simulink model "GuidanceLaw"  (R2023b)
settings: Solver=ode4  StartTime=0.0  StopTime=400  FixedStep=0.05  RelTol=1e-3
values from neighbouring files (symbols this model uses):
  APCMD_TYPE : value not decoded    [apDataDictionary.sldd]
  missionRoutePlan_struct = struct(      'validWpNum_u8', uint8(5),      'missionRoute_struct', repmat(wpDefault_struct, double(maxWpNum_u8), 1))    [initMissionRoutePlan_MC.m]
  MSSN_TYPE : value not decoded    [apDataDictionary.sldd]
  setPoint_struct = struct('lat_deg_d',double(31.200000),'lon_deg_d',double(121.500000),'alt_m_f',single(100),'yaw_deg_f',single(0))    [APTest.m]
undefined symbols (not defined in the file or in its folder): apParams
libraries: simulink x13, simulink_extras x3
(part 4 of 7)

== matlab function GuidanceLaw/Subsystem/wpMssnHandle/GuiLaw/guiLawSelect/guiLawSelect ==
  data: flightPhase_enum input; guiLawType_u8 output; fwL1LineGui_b output; fwL1CirGui_b output; fwAirSpdGui_b output; fwVertSpdGui_b output; mcSpdGui_b output; yawGui_b output; preWp_struct input; curWp_struct input; segMssnType_u8 output; tiltEnable_b output
function [guiLawType_u8, fwL1LineGui_b, fwL1CirGui_b, fwAirSpdGui_b, fwVertSpdGui_b, mcSpdGui_b, yawGui_b, segMssnType_u8, tiltEnable_b] = guiLawSelect(flightPhase_enum, ...
    preWp_struct, curWp_struct)
%#codegen
%
% 功能：
% 根据当前飞行阶段、上一航点类型和当前航点类型选择导引律。
%
% 当前执行航段定义：
% preWp_struct -> curWp_struct
%
% segMssnType_u8:
% 0：无效，1：旋翼垂直起飞，2：旋翼直线，3：旋翼垂直降落，4：旋翼前倾，5：固定翼后倾，6：固定翼直线，7：固定翼圆弧

%% 获取航点类型

preWpType_u8 = preWp_struct.wpType_u8;
curWpType_u8 = curWp_struct.wpType_u8;

%% 默认关闭所有导引律

guiLawType_u8 = uint8(0);
fwL1LineGui_b = false;
fwL1CirGui_b = false;
fwAirSpdGui_b = false;
fwVertSpdGui_b = false;
mcSpdGui_b = false;
yawGui_b = false;
segMssnType_u8 = uint8(0);    % 航段任务类型无效
tiltEnable_b = false;       % 倾转使能标志

%% 根据上一航点和当前航点判断判断
% 当前是垂直起飞航点
if curWpType_u8 == WP_TYPE.MC_TAKEOFF_WP
    % 旋翼速度导引、偏航角导引使能
    mcSpdGui_b = true;
    yawGui_b = true;
    guiLawType_u8 = uint8(1);
    segMssnType_u8 = uint8(1);        % 航段任务类型为旋翼垂直起飞
    tiltEnable_b = false;

% 当前是旋翼直线航点
elseif (preWpType_u8 == WP_TYPE.MC_TAKEOFF_WP && curWpType_u8 == WP_TYPE.MC_LINE_WP) || ...
        (preWpType_u8 == WP_TYPE.FW_LINE_WP && curWpType_u8 == WP_TYPE.MC_LINE_WP)||...
        (preWpType_u8 == WP_TYPE.MC_LINE_WP && curWpType_u8 == WP_TYPE.MC_LINE_WP)
    switch flightPhase_enum
        case FLIGHT_PHASE.MC_FLIGHT
            % 旋翼速度导引、偏航角导引使能
            mcSpdGui_b = true;
            yawGui_b = true;
            guiLawType_u8 = uint8(1);
            segMssnType_u8 = uint8(2);        % 航段任务类型为旋翼直线

        case FLIGHT_PHASE.TILT_FLIGHT
            % L1直线导引、fw空速导引、fw垂速导引、偏航角导引使能
            fwL1LineGui_b = true;
            fwAirSpdGui_b = true;
            fwVertSpdGui_b = true;
            yawGui_b = true;
            guiLawType_u8 = uint8(2);
            segMssnType_u8 = uint8(5);        % 航段任务类型为固定翼后倾

        case FLIGHT_PHASE.FW_FLIGHT
            % L1直线导引、fw空速导引、fw垂速导引使能
            fwL1LineGui_b = true;
            fwAirSpdGui_b = true;
            fwVertSpdGui_b = true;
            guiLawType_u8 = uint8(3);
            segMssnType_u8 = uint8(5);        % 航段任务类型为固定翼后倾

        otherwise
            % 不处理
    end
    tiltEnable_b = false;

% 当前是垂直降落航点
elseif (preWpType_u8 == WP_TYPE.MC_TAKEOFF_WP && curWpType_u8 == WP_TYPE.MC_LAND_WP) || (preWpType_u8 == WP_TYPE.FW_LINE_WP && curWpType_u8 == WP_TYPE.MC_LAND_WP)||...
        (preWpType_u8 == WP_TYPE.MC_LINE_WP && curWpType_u8 == WP_TYPE.MC_LAND_WP) || (preWpType_u8 == WP_TYPE.MC_LAND_WP && curWpType_u8 == WP_TYPE.MC_LAND_WP)
    switch flightPhase_enum
        case {FLIGHT_PHASE.MC_FLIGHT, FLIGHT_PHASE.MC_GROUND}
            % 旋翼速度导引、偏航角导引使能
            mcSpdGui_b = true;
            yawGui_b = true;
            guiLawType_u8 = uint8(1);

            if preWpType_u8 == WP_TYPE.MC_LAND_WP && curWpType_u8 == WP_TYPE.MC_LAND_WP
                segMssnType_u8 = uint8(3);        % 航段任务类型为旋翼垂直着陆
            else
                segMssnType_u8 = uint8(2);        % 航段任务类型为旋翼直线
            end

        case FLIGHT_PHASE.TILT_FLIGHT
            % L1直线导引、fw空速导引、fw垂速导引、偏航角导引使能
            fwL1LineGui_b = true;
            fwAirSpdGui_b = true;
            fwVertSpdGui_b = true;
            yawGui_b = true;
            guiLawType_u8 = uint8(2);
            segMssnType_u8 = uint8(5);        % 航段任务类型为固定翼后倾

        case FLIGHT_PHASE.FW_FLIGHT
            % L1直线导引、fw空速导引、fw垂速导引使能
            fwL1LineGui_b = true;
            fwAirSpdGui_b = true;
            fwVertSpdGui_b = true;
            guiLawType_u8 = uint8(3);
            segMssnType_u8 = uint8(5);        % 航段任务类型为固定翼后倾

        otherwise
            % 不处理
    end
    tiltEnable_b = false;
    
% 当前是固定翼直线航点
elseif (preWpType_u8 == WP_TYPE.MC_TAKEOFF_WP && curWpType_u8 == WP_TYPE.FW_LINE_WP) || (preWpType_u8 == WP_TYPE.MC_LINE_WP && curWpType_u8 == WP_TYPE.FW_LINE_WP)||...
        (preWpType_u8 == WP_TYPE.FW_LINE_WP && curWpType_u8 == WP_TYPE.FW_LINE_WP)
    switch flightPhase_enum
        case {FLIGHT_PHASE.MC_FLIGHT, FLIGHT_PHASE.TILT_FLIGHT}
            % L1直线导引、fw空速导引、fw垂速导引、偏航角导引使能
            fwL1LineGui_b = true;
            fwAirSpdGui_b = true;
            fwVertSpdGui_b = true;
            yawGui_b = true;
            guiLawType_u8 = uint8(2);
            segMssnType_u8 = uint8(4);        % 航段任务类型为旋翼前倾

        case FLIGHT_PHASE.FW_FLIGHT
            % L1直线导引、fw空速导引、fw垂速导引使能
            fwL1LineGui_b = true;
            fwAirSpdGui_b = true;
            fwVertSpdGui_b = true;
            guiLawType_u8 = uint8(3);
            segMssnType_u8 = uint8(6);        % 航段任务类型为固定翼直线

        otherwise
            % 不处理
    end
    tiltEnable_b = true;

% 当前是圆弧航点
elseif curWpType_u8 == WP_TYPE.FW_CIR_WP
    % L1圆弧导引、fw空速导引、fw垂速导引使能
    fwL1CirGui_b = true;
    fwAirSpdGui_b = true;
    fwVertSpdGui_b = true;
    guiLawType_u8 = uint8(4);
    tiltEnable_b = true;
    segMssnType_u8 = uint8(7);        % 航段任务类型为固定翼圆弧

else
    % 不处理
end

end

== matlab function GuidanceLaw/Subsystem/wpMssnHandle/GuiLaw/fwAirSpdGuidance/fwAirSpdGuidance ==
  data: curPosNEU_m_f input; curAirSpd_mps_f input; velNEU_mps_f input; preWp_struct input; speedCmd_mps_f output; curWp_struct input; dt_s_f input; reset_b input; param_f input; segMssnType_u8 input; mssnType_u8 input
function speedCmd_mps_f = fwAirSpdGuidance(curPosNEU_m_f, curAirSpd_mps_f, velNEU_mps_f, preWp_struct, curWp_struct, dt_s_f, reset_b, param_f, segMssnType_u8, mssnType_u8)
%#codegen
%
% 速度指令生成导引算法
%
% 功能：
% 1. 前倾和固定翼飞行阶段生成等效空速指令；
% 2. 后倾阶段生成水平地速指令；
% 3. 普通自动后倾根据目标点剩余沿程距离生成减速包线；
% 4. 自动着陆定向后倾进入航段后立即按设定减速度降低水平速度；
% 5. 定向后倾目标点只用于航向/航迹锚定，不参与速度指令计算；
% 6. 后倾速度降至旋翼阶段准入速度后，由外部切换至旋翼导引律。
%
% param_f定义：
% 1  minOptAirspeed_mps_f          正常固定翼最小空速，m/s；
% 2  maxOptAirSpeed_mps_f          最大速度，m/s；
% 3  cruiseAirspeed_mps_f          默认巡航空速，m/s；
% 4  airspeedAccelMax_mps2_f       空速指令最大增加率，m/s^2；
% 5  airspeedDecelMax_mps2_f       空速指令最大减小率，m/s^2；
% 6  backTransDecel_mps2_f         后倾期望水平减速度，m/s^2；
% 7  backTransAnchorRadius_m_f     普通自动后倾减速包线锚定半径，m；
% 8  backTransFastAnchorSpd_mps_f  普通自动后倾快速过点虚拟末速度，m/s；
%                                  同时作为定向后倾目标水平速度，m/s。
%
% 注意：
% 当该函数用于自动着陆定向后倾时，param_f(8)应低于外部MC_FLIGHT
% 准入速度，并留有适当裕度。
% 当前简化六自由度模型在水平速度不大于10 m/s时进入MC_FLIGHT，
% 因此建议本参数使用7~8 m/s。

persistent initialized_b
persistent backTransLast_b
% persistent directionBackTiltLast_b
persistent speedCmdState_mps_f

if isempty(initialized_b)
    initialized_b = false;
    backTransLast_b = false;
    % directionBackTiltLast_b = false;
    speedCmdState_mps_f = single(0.0);
end

%% 1. 参数解析

minOptAirspeed_mps_f = max(param_f(1), single(0.0));
maxOptAirspeed_mps_f = max(param_f(2), minOptAirspeed_mps_f);

cruiseAirspeed_mps_f = max(param_f(3), single(0.0));

airspeedAccelMax_mps2_f = max(param_f(4), single(0.0));
airspeedDecelMax_mps2_f = max(param_f(5), single(0.0));

backTransDecel_mps2_f = max(param_f(6), single(0.1));
backTransAnchorRadius_m_f = max(param_f(7), single(0.0));
backTransFastAnchorSpd_mps_f = max(param_f(8), single(0.0));

% 定向后倾复用param_f(8)作为目标水平速度。该速度允许低于正常固定翼
% 最小空速，因为后倾过程中旋翼升力逐步接管。
% directionBackTiltTargetSpd_mps_f = constrain_scalar(max(param_f(8), single(0.0)), single(0.0), maxOptAirspeed_mps_f);

dtUse_s_f = max(dt_s_f, single(0.0));

%% 2. 判断速度导引模式

isBackTransition_b = segMssnType_u8 == uint8(5);        % 后倾航段任务
isDirectionBackTilt_b = isBackTransition_b && mssnType_u8 == MSSN_TYPE.AUTO_LAND_DIRECTION_BACK_TILT;

speedModeChanged_b = isBackTransition_b ~= backTransLast_b; %|| isDirectionBackTilt_b ~= directionBackTiltLast_b;

%% 3. 正常固定翼空速导引

if ~isBackTransition_b

    airSpdPlan_mps_f = curWp_struct.spd_mps_f;

    if airSpdPlan_mps_f > single(0.0)
        speedBase_mps_f = airSpdPlan_mps_f;
    else
        speedBase_mps_f = cruiseAirspeed_mps_f;
    end

    speedRaw_mps_f = constrain_scalar(speedBase_mps_f, minOptAirspeed_mps_f, maxOptAirspeed_mps_f);

    if reset_b || ~initialized_b || speedModeChanged_b

        % 从当前实际空速无跳变接入正常固定翼空速导引。
        speedCmdState_mps_f = constrain_scalar(curAirSpd_mps_f, minOptAirspeed_mps_f, maxOptAirspeed_mps_f);

        initialized_b = true;

    else

        speedCmdState_mps_f = rateLimit(speedRaw_mps_f, speedCmdState_mps_f, airspeedAccelMax_mps2_f, airspeedDecelMax_mps2_f, dtUse_s_f);

        speedCmdState_mps_f = constrain_scalar(speedCmdState_mps_f, minOptAirspeed_mps_f, maxOptAirspeed_mps_f);

    end

%% 4. 后倾阶段水平地速导引

else

    %% 4.1 计算当前水平地速

    groundSpdSq_m2ps2_f = velNEU_mps_f(1) * velNEU_mps_f(1) + velNEU_mps_f(2) * velNEU_mps_f(2);

    groundSpd_mps_f = sqrt(max(groundSpdSq_m2ps2_f, single(0.0)));

    if isDirectionBackTilt_b

        %% 4.2 自动着陆定向后倾：进入航段后立即减速

        if reset_b || ~initialized_b || speedModeChanged_b

            % 从当前实际水平地速无跳变接入。
            speedCmdState_mps_f = constrain_scalar(groundSpd_mps_f, single(0.0), maxOptAirspeed_mps_f);

            initialized_b = true;

        else

            % 不计算锚点距离。锚点只供横向航迹导引使用。
            speedCmdState_mps_f = rateLimit(single(0), speedCmdState_mps_f, single(0.0), backTransDecel_mps2_f, dtUse_s_f);

            % 定向后倾阶段不施加正常固定翼最小空速下限。
            speedCmdState_mps_f = constrain_scalar(speedCmdState_mps_f, single(0), maxOptAirspeed_mps_f);

        end

    else

        %% 4.3 普通自动后倾：保留原来的距离减速包线

        %% 4.3.1 计算水平航段向量

        pathVectorN_m_f = curWp_struct.posN_m_f - preWp_struct.posN_m_f;
        pathVectorE_m_f = curWp_struct.posE_m_f - preWp_struct.posE_m_f;

        pathLengthSq_m2_f = pathVectorN_m_f * pathVectorN_m_f + pathVectorE_m_f * pathVectorE_m_f;

        pathLength_m_f = sqrt(max(pathLengthSq_m2_f, single(0.0)));

        %% 4.3.2 计算当前位置到目标航点的向量

        targetVectorN_m_f = curWp_struct.posN_m_f - curPosNEU_m_f(1);
        targetVectorE_m_f = curWp_struct.posE_m_f - curPosNEU_m_f(2);

        targetDistSq_m2_f = targetVectorN_m_f * targetVectorN_m_f + targetVectorE_m_f * targetVectorE_m_f;

        targetDist_m_f = sqrt(max(targetDistSq_m2_f, single(0.0)));

        %% 4.3.3 计算剩余沿程距离

        if pathLength_m_f > single(0.1)

            pathTangentN_f = pathVectorN_m_f / pathLength_m_f;
            pathTangentE_f = pathVectorE_m_f / pathLength_m_f;

            remainAlongTrack_m_f = targetVectorN_m_f * pathTangentN_f + targetVectorE_m_f * pathTangentE_f;

        else

            remainAlongTrack_m_f = targetDist_m_f;

        end

        remainAlongTrack_m_f = max(remainAlongTrack_m_f, single(0.0));

        %% 4.3.4 确定普通自动后倾虚拟末速度

        if curWp_struct.fastWp_b
            speedAnchor_mps_f = backTransFastAnchorSpd_mps_f;       % 这里给了个旋翼最大巡航速度
        else
            speedAnchor_mps_f = single(0.0);
        end

        %% 4.3.5 根据剩余距离反算速度包线

        effectiveRemainDist_m_f = remainAlongTrack_m_f - backTransAnchorRadius_m_f;

        effectiveRemainDist_m_f = max(effectiveRemainDist_m_f, single(0.0));

        envelopeSpdSq_m2ps2_f = speedAnchor_mps_f * speedAnchor_mps_f + single(2.0) * backTransDecel_mps2_f * effectiveRemainDist_m_f;

        groundSpdEnvelopeRaw_mps_f = sqrt(max(envelopeSpdSq_m2ps2_f, single(0.0)));

        groundSpdEnvelope_mps_f = constrain_scalar(groundSpdEnvelopeRaw_mps_f, minOptAirspeed_mps_f, maxOptAirspeed_mps_f);

        %% 4.3.6 更新普通自动后倾速度指令

        if reset_b || ~initialized_b || speedModeChanged_b

            speedCmdState_mps_f = constrain_scalar(groundSpd_mps_f, minOptAirspeed_mps_f, maxOptAirspeed_mps_f);

            initialized_b = true;

        else

            speedRaw_mps_f = min(speedCmdState_mps_f, groundSpdEnvelope_mps_f);

            speedCmdState_mps_f = rateLimit(speedRaw_mps_f, speedCmdState_mps_f, single(0.0), backTransDecel_mps2_f, dtUse_s_f);

            speedCmdState_mps_f = constrain_scalar(speedCmdState_mps_f, minOptAirspeed_mps_f, maxOptAirspeed_mps_f);

        end

    end

end


%% 5. 输出及模式记录

speedCmd_mps_f = speedCmdState_mps_f;

backTransLast_b = isBackTransition_b;
% directionBackTiltLast_b = isDirectionBackTilt_b;

end

== matlab function GuidanceLaw/Subsystem/wpMssnHandle/GuiLaw/fwAirSpdGuidance/fwAirSpdGuidance1 ==
  data: curPosNEU_m_f input; curAirSpd_mps_f input; velNEU_mps_f input; preWp_struct input; speedCmd_mps_f output; curWp_struct input; dt_s_f input; reset_b input; param_f input; segMssnType_u8 input
function speedCmd_mps_f = fwAirSpdGuidance(curPosNEU_m_f, curAirSpd_mps_f, velNEU_mps_f, preWp_struct, curWp_struct, dt_s_f, reset_b, param_f, segMssnType_u8)
%#codegen
%
% 速度指令生成导引算法
%
% 功能：
% 1. 前倾和固定翼飞行阶段生成等效空速指令；
% 2. 后倾阶段生成水平地速指令；
% 3. 后倾阶段根据剩余沿程距离反算允许水平地速；
% 4. 快速过点采用非零虚拟末速度构造减速包线；
% 5. 减速悬停采用零虚拟末速度构造减速包线；
% 6. 完成旋翼构型转换后，由外部切换至旋翼导引律。
%
% param_f定义：
% 1  minOptAirspeed_mps_f          最小空速，m/s；
% 2  maxOptAirSpeed_mps_f          最大速度，m/s；
% 3  cruiseAirspeed_mps_f          默认巡航空速，m/s；
% 4  airspeedAccelMax_mps2_f       空速指令最大增加率，m/s^2；
% 5  airspeedDecelMax_mps2_f       空速指令最大减小率，m/s^2；
% 6  backTransDecel_mps2_f         后倾期望水平减速度，m/s^2；
% 7  backTransAnchorRadius_m_f     后倾减速包线锚定半径，m；
% 8  backTransFastAnchorSpd_mps_f  快速过点虚拟末速度锚点，m/s。

persistent initialized_b
persistent backTransLast_b
persistent speedCmdState_mps_f

if isempty(initialized_b)
    initialized_b = false;
    backTransLast_b = false;
    speedCmdState_mps_f = single(0.0);
end

%% 1. 参数解析

minOptAirspeed_mps_f = max(param_f(1), single(0.0));
maxOptAirspeed_mps_f = max(param_f(2), minOptAirspeed_mps_f);

cruiseAirspeed_mps_f = max(param_f(3), single(0.0));

airspeedAccelMax_mps2_f = max(param_f(4), single(0.0));
airspeedDecelMax_mps2_f = max(param_f(5), single(0.0));

backTransDecel_mps2_f = max(param_f(6), single(0.1));
backTransAnchorRadius_m_f = max(param_f(7), single(0.0));
backTransFastAnchorSpd_mps_f = max(param_f(8), single(0.0));

dtUse_s_f = max(dt_s_f, single(0.0));

%% 2. 判断速度导引模式

isBackTransition_b = segMssnType_u8 == uint8(5);
speedModeChanged_b = isBackTransition_b ~= backTransLast_b;

%% 3. 正常固定翼空速导引

if ~isBackTransition_b

    airSpdPlan_mps_f = curWp_struct.spd_mps_f;

    if airSpdPlan_mps_f > single(0.0)
        speedBase_mps_f = airSpdPlan_mps_f;
    else
        speedBase_mps_f = cruiseAirspeed_mps_f;
    end

    speedRaw_mps_f = constrain_scalar(speedBase_mps_f, minOptAirspeed_mps_f, maxOptAirspeed_mps_f);

    if reset_b || ~initialized_b || speedModeChanged_b

        % 从当前实际空速接入固定翼空速导引。
        speedCmdState_mps_f = constrain_scalar(curAirSpd_mps_f, minOptAirspeed_mps_f, maxOptAirspeed_mps_f);
        initialized_b = true;

    else

        speedCmdState_mps_f = rateLimit(speedRaw_mps_f, speedCmdState_mps_f, airspeedAccelMax_mps2_f, airspeedDecelMax_mps2_f, dtUse_s_f);

        speedCmdState_mps_f = constrain_scalar(speedCmdState_mps_f, minOptAirspeed_mps_f, maxOptAirspeed_mps_f);

    end

%% 4. 后倾阶段水平地速导引

else

    %% 4.1 计算当前水平地速

    groundSpdSq_m2ps2_f = velNEU_mps_f(1) * velNEU_mps_f(1) + velNEU_mps_f(2) * velNEU_mps_f(2);

    groundSpd_mps_f = sqrt(max(groundSpdSq_m2ps2_f, single(0.0)));

    %% 4.2 计算水平航段向量

    pathVectorN_m_f = curWp_struct.posN_m_f - preWp_struct.posN_m_f;
    pathVectorE_m_f = curWp_struct.posE_m_f - preWp_struct.posE_m_f;

    pathLengthSq_m2_f = pathVectorN_m_f * pathVectorN_m_f + pathVectorE_m_f * pathVectorE_m_f;

    pathLength_m_f = sqrt(max(pathLengthSq_m2_f, single(0.0)));

    %% 4.3 计算当前位置到目标航点的向量

    targetVectorN_m_f = curWp_struct.posN_m_f - curPosNEU_m_f(1);
    targetVectorE_m_f = curWp_struct.posE_m_f - curPosNEU_m_f(2);

    targetDistSq_m2_f = targetVectorN_m_f * targetVectorN_m_f + targetVectorE_m_f * targetVectorE_m_f;

    targetDist_m_f = sqrt(max(targetDistSq_m2_f, single(0.0)));

    %% 4.4 计算剩余沿程距离

    if pathLength_m_f > single(0.5)

        pathTangentN_f = pathVectorN_m_f / pathLength_m_f;
        pathTangentE_f = pathVectorE_m_f / pathLength_m_f;

        remainAlongTrack_m_f = targetVectorN_m_f * pathTangentN_f + targetVectorE_m_f * pathTangentE_f;

    else

        % 航段长度过小时退化为目标点直线距离。
        remainAlongTrack_m_f = targetDist_m_f;

    end

    remainAlongTrack_m_f = max(remainAlongTrack_m_f, single(0.0));

    %% 4.5 确定虚拟末速度锚点

    if curWp_struct.fastWp_b
    
        % 非零虚拟末速度锚点。
        speedAnchor_mps_f = backTransFastAnchorSpd_mps_f;
    
    else
    
        % 零虚拟末速度锚点。
        speedAnchor_mps_f = single(0.0);
    
    end

    %% 4.6 根据剩余距离反算速度包线

    effectiveRemainDist_m_f = remainAlongTrack_m_f - backTransAnchorRadius_m_f;

    effectiveRemainDist_m_f = max(effectiveRemainDist_m_f, single(0.0));

    envelopeSpdSq_m2ps2_f = speedAnchor_mps_f * speedAnchor_mps_f + single(2.0) * backTransDecel_mps2_f * effectiveRemainDist_m_f;

    groundSpdEnvelopeRaw_mps_f = sqrt(max(envelopeSpdSq_m2ps2_f, single(0.0)));

    groundSpdEnvelope_mps_f = constrain_scalar(groundSpdEnvelopeRaw_mps_f, minOptAirspeed_mps_f, maxOptAirspeed_mps_f);

    %% 4.7 更新后倾速度指令状态

    if reset_b || ~initialized_b || speedModeChanged_b
    
        speedCmdState_mps_f = constrain_scalar(groundSpd_mps_f, minOptAirspeed_mps_f, maxOptAirspeed_mps_f);
    
        initialized_b = true;
    
    else
    
        speedRaw_mps_f = min(speedCmdState_mps_f, groundSpdEnvelope_mps_f);
    
        speedCmdState_mps_f = rateLimit(speedRaw_mps_f, speedCmdState_mps_f, single(0.0), backTransDecel_mps2_f, dtUse_s_f);
    
        speedCmdState_mps_f = constrain_scalar(speedCmdState_mps_f, minOptAirspeed_mps_f, maxOptAirspeed_mps_f);
    
    end

end

%% 5. 输出及模式记录

speedCmd_mps_f = speedCmdState_mps_f;

backTransLast_b = isBackTransition_b;

end

== matlab function GuidanceLaw/Subsystem/wpMssnHandle/GuiLaw/mcSpdGuidance/mcTrajectoryGeneratorNEU/TrajectoryGeneratorNEU1 ==
  data: trajPosNEU_m_f output; curPosNEU_m_f input; curVelNEU_mps_f input; curAccNEU_mps2_f input; preWpNEU_m_f input; curWpNEU_m_f input; nextWpNEU_m_f input; velSpNEU_mps_f input; posVelValid_vec input; isHoverWp_b input; forceStop_b input; segSwitch_b input; newOriOldNEU_m_f input; dt_s_f input; reset_b input; paramNE_f input; trajVelNEU_mps_f output; trajAccNEU_mps2_f output; trajJerkNEU_mps3_f output; paramU_f input
function [trajPosNEU_m_f, trajVelNEU_mps_f, trajAccNEU_mps2_f, trajJerkNEU_mps3_f] = trajGeneratorNEU(curPosNEU_m_f, curVelNEU_mps_f, curAccNEU_mps2_f, preWpNEU_m_f, curWpNEU_m_f, nextWpNEU_m_f, ...
    velSpNEU_mps_f, posVelValid_vec, isHoverWp_b, forceStop_b, segSwitch_b, newOriOldNEU_m_f, dt_s_f, reset_b, paramNE_f, paramU_f)
%#codegen
%
% 功能：
% 生成NEU三轴jerk受限平滑轨迹，并进行N/E/U三轴S曲线时间同步。
%
% velSpNEU_mps_f：
% 1. 对应位置无效时，为纯速度目标；
% 2. 对应位置有效时，为位置导引速度上的速度前馈。
%
% posVelValid_vec：[posNEValid; velNEValid; posUValid; velUValid]
%
% paramNE_f：
% 1 最大水平jerk，[m/s^3]
% 2 最大水平加速度，[m/s^2]
% 3 最大水平速度，[m/s]
% 4 水平巡航速度，[m/s]
% 5 最大允许水平轨迹误差，[m]
% 6 水平航点接受半径，[m]
% 7 最小前视距离，[m]
% 8 转弯判断最小轨迹速度，[m/s]
% 9 转弯判断方向余弦阈值
% 10 前倾转换阶段旋翼水平速度，[m/s]
%
% paramU_f：
% 1 最大垂向jerk，[m/s^3]
% 2 爬升轨迹使用的最大垂向加速度幅值，[m/s^2]
% 3 下降轨迹使用的最大垂向加速度幅值，[m/s^2]
% 4 最大爬升速度，[m/s]
% 5 最大下降速度幅值，[m/s]
% 6 最大允许垂向轨迹误差，[m]
% 7 垂向航点接受半径，[m]
%
% 垂向非对称约束：
% 1. 根据未平滑垂向速度目标rawVelSpNEU_mps_f(3)的方向，选择一整套
%    垂向速度和加速度幅值约束；
% 2. 选定后，单轴S曲线规划器内部仍使用对称的+/-maxAcceleration约束；
% 3. rawVelSpU为0时保持上一套约束，避免停车附近反复切换。

%% 常量

smallValue_f = single(1.0e-6);
floatEpsilon_f = single(1.1920929e-7);
clampAccuracy_mps_f = single(0.5);

%% 最小持久状态
% 轨迹生成器每个周期都会根据当前状态重新规划S曲线，并在同一周期推进dt。
persistent trajAccStateNEU_mps2_f trajVelStateNEU_mps_f trajPosStateNEU_m_f
persistent selectedUConstraintModeState_i8
persistent previousMaxSpeedNEState_mps_f
persistent initialized_b

if isempty(initialized_b)
    initialized_b = false;

    trajAccStateNEU_mps2_f = single(zeros(3,1));
    trajVelStateNEU_mps_f = single(zeros(3,1));
    trajPosStateNEU_m_f = single(zeros(3,1));
    selectedUConstraintModeState_i8 = int8(0);
    previousMaxSpeedNEState_mps_f = single(0.0);
else
    initialized_b = true;
end

%% 参数读取
maxJerkNE_mps3_f = max(paramNE_f(1), smallValue_f);
maxAccNE_mps2_f = max(paramNE_f(2), smallValue_f);
maxVelNE_mps_f = max(paramNE_f(3), smallValue_f);
cruiseSpeedNE_mps_f = constrain_scalar(paramNE_f(4), single(0.0), maxVelNE_mps_f);
maxTrajErrorNE_m_f = max(paramNE_f(5), smallValue_f);
horizonAptRadius_m_f = max(paramNE_f(6), smallValue_f);
minLookaheadDist_m_f = max(paramNE_f(7), horizonAptRadius_m_f);
turnMinSpeed_mps_f = max(paramNE_f(8), single(0.0));
turnCosThreshold_f = constrain_scalar(paramNE_f(9), single(-1.0), single(1.0));
fwdFixedSpd_mps_f = max(paramNE_f(10), smallValue_f);

maxJerkU_mps3_f = max(paramU_f(1), smallValue_f);
maxAccUp_mps2_f = max(paramU_f(2), smallValue_f);
maxAccDown_mps2_f = max(paramU_f(3), smallValue_f);
maxVelUp_mps_f = max(paramU_f(4), smallValue_f);
maxVelDown_mps_f = max(paramU_f(5), smallValue_f);
maxTrajErrorU_m_f = max(paramU_f(6), smallValue_f);
verticalAcceptanceRadius_m_f = max(paramU_f(7), smallValue_f);

axisMaxJerkNEU_mps3_f = single([maxJerkNE_mps3_f; maxJerkNE_mps3_f; maxJerkU_mps3_f]);

dtEff_s_f = max(dt_s_f, single(0.0));

%% 输入有效性
posNEValid_b = logical(posVelValid_vec(1));
velNEValid_b = logical(posVelValid_vec(2));
posUValid_b = logical(posVelValid_vec(3));
velUValid_b = logical(posVelValid_vec(4));

%% 初始化、复位或航段坐标系切换
if reset_b || ~initialized_b
    trajAccStateNEU_mps2_f = curAccNEU_mps2_f;
    trajVelStateNEU_mps_f = curVelNEU_mps_f;
    trajPosStateNEU_m_f = curPosNEU_m_f;

    trajAccStateNEU_mps2_f(1) = constrain_scalar(curAccNEU_mps2_f(1), -maxAccNE_mps2_f, maxAccNE_mps2_f);
    trajAccStateNEU_mps2_f(2) = constrain_scalar(curAccNEU_mps2_f(2), -maxAccNE_mps2_f, maxAccNE_mps2_f);
    trajAccStateNEU_mps2_f(3) = constrain_scalar(curAccNEU_mps2_f(3), -maxAccDown_mps2_f, maxAccUp_mps2_f);

    trajVelStateNEU_mps_f(1) = constrain_scalar(curVelNEU_mps_f(1), -maxVelNE_mps_f, maxVelNE_mps_f);
    trajVelStateNEU_mps_f(2) = constrain_scalar(curVelNEU_mps_f(2), -maxVelNE_mps_f, maxVelNE_mps_f);
    trajVelStateNEU_mps_f(3) = constrain_scalar(curVelNEU_mps_f(3), -maxVelDown_mps_f, maxVelUp_mps_f);

    % 1表示爬升约束，-1表示下降约束，0表示尚未选择方向并采用保守值。
    if curVelNEU_mps_f(3) > smallValue_f
        selectedUConstraintModeState_i8 = int8(1);
    elseif curVelNEU_mps_f(3) < -smallValue_f
        selectedUConstraintModeState_i8 = int8(-1);
    else
        selectedUConstraintModeState_i8 = int8(0);
    end

    previousMaxSpeedNEState_mps_f = single(0.0);

elseif segSwitch_b
    % 各航段坐标轴方向不变，仅平移原点
    trajPosStateNEU_m_f = trajPosStateNEU_m_f - newOriOldNEU_m_f;
else
    % 不处理
end

%% 按有效性组合生成原始速度目标

% 先装载速度输入。位置有效时，它是位置速度的前馈；位置无效时，
% 它就是直接送给S曲线平滑器的纯速度目标。无效速度分量保持为0。
rawVelSpNEU_mps_f = single(zeros(3,1));

if velNEValid_b
    rawVelSpNEU_mps_f(1:2) = velSpNEU_mps_f(1:2);
end

if velUValid_b
    rawVelSpNEU_mps_f(3) = velSpNEU_mps_f(3);
end

if forceStop_b
    % 强制停车优先级最高，忽略位置目标和速度前馈。
    rawVelSpNEU_mps_f = single(zeros(3,1));

elseif posNEValid_b && posUValid_b
    %% NE和U位置同时有效：生成三维位置速度目标
    waypointsNEU_m_f = [preWpNEU_m_f, curWpNEU_m_f, nextWpNEU_m_f];

    [crossingPointNEU_m_f, targetSpeedNE_mps_f, previousMaxSpeedNEState_mps_f] = get_xy_guidance_constraints_handle(trajPosStateNEU_m_f, trajVelStateNEU_mps_f, waypointsNEU_m_f, ...
        isHoverWp_b, cruiseSpeedNE_mps_f, maxJerkNE_mps3_f, maxAccNE_mps2_f, horizonAptRadius_m_f, minLookaheadDist_m_f, turnMinSpeed_mps_f, ...
        turnCosThreshold_f, previousMaxSpeedNEState_mps_f, smallValue_f);

    if isHoverWp_b
        nextWpForUSpeed_m_f = curWpNEU_m_f(3);
    else
        nextWpForUSpeed_m_f = nextWpNEU_m_f(3);
    end

    maxAllowedSpeedU_mps_f = get_max_z_speed_handle(trajPosStateNEU_m_f(3), curWpNEU_m_f(3), nextWpForUSpeed_m_f, maxJerkU_mps3_f, maxAccUp_mps2_f, maxAccDown_mps2_f, ...
        maxVelUp_mps_f, maxVelDown_mps_f, verticalAcceptanceRadius_m_f, smallValue_f);

    posToCrossingNEU_m_f = crossingPointNEU_m_f - trajPosStateNEU_m_f;
    directionToCrossingNEU_f = unit_or_zero(posToCrossingNEU_m_f, smallValue_f);
    combinedSpeed_mps_f = sqrt(targetSpeedNE_mps_f * targetSpeedNE_mps_f + maxAllowedSpeedU_mps_f * maxAllowedSpeedU_mps_f);
    posVelSpNEU_mps_f = directionToCrossingNEU_f * combinedSpeed_mps_f;

    % 先限制水平模长，再限制垂向模长。
    % 0.5是小速度区间判定精度accuracy，不是另一方向的固定缩放系数。
    posVelSpNEU_mps_f = clamp_to_xy_norm(posVelSpNEU_mps_f, targetSpeedNE_mps_f, clampAccuracy_mps_f, floatEpsilon_f);
    posVelSpNEU_mps_f = clamp_to_u_norm(posVelSpNEU_mps_f, maxAllowedSpeedU_mps_f, clampAccuracy_mps_f, floatEpsilon_f);

    if velNEValid_b
        rawVelSpNEU_mps_f(1:2) = rawVelSpNEU_mps_f(1:2) + posVelSpNEU_mps_f(1:2);
    else
        rawVelSpNEU_mps_f(1:2) = posVelSpNEU_mps_f(1:2);
    end

    if velUValid_b
        rawVelSpNEU_mps_f(3) = rawVelSpNEU_mps_f(3) + posVelSpNEU_mps_f(3);
    else
        rawVelSpNEU_mps_f(3) = posVelSpNEU_mps_f(3);
    end

elseif posNEValid_b
    %% 仅NE位置有效：生成二维水平位置速度目标
    waypointsNEU_m_f = [preWpNEU_m_f, curWpNEU_m_f, nextWpNEU_m_f];

    [crossingPointNEU_m_f, targetSpeedNE_mps_f, previousMaxSpeedNEState_mps_f] = get_xy_guidance_constraints_handle(trajPosStateNEU_m_f, trajVelStateNEU_mps_f, waypointsNEU_m_f, ...
        isHoverWp_b, cruiseSpeedNE_mps_f, maxJerkNE_mps3_f, maxAccNE_mps2_f, horizonAptRadius_m_f, minLookaheadDist_m_f, turnMinSpeed_mps_f, ...
        turnCosThreshold_f, previousMaxSpeedNEState_mps_f, smallValue_f);

    posToCrossingNE_m_f = crossingPointNEU_m_f(1:2) - trajPosStateNEU_m_f(1:2);
    directionToCrossingNE_f = unit_or_zero(posToCrossingNE_m_f, smallValue_f);
    posVelSpNE_mps_f = directionToCrossingNE_f * targetSpeedNE_mps_f;

    if velNEValid_b
        rawVelSpNEU_mps_f(1:2) = rawVelSpNEU_mps_f(1:2) + posVelSpNE_mps_f;
    else
        rawVelSpNEU_mps_f(1:2) = posVelSpNE_mps_f;
    end

elseif posUValid_b
    %% 仅U位置有效：生成一维垂向位置速度目标
    if isHoverWp_b
        nextWpForUSpeed_m_f = curWpNEU_m_f(3);
    else
        nextWpForUSpeed_m_f = nextWpNEU_m_f(3);
    end

    maxAllowedSpeedU_mps_f = get_max_z_speed_handle(trajPosStateNEU_m_f(3), curWpNEU_m_f(3), nextWpForUSpeed_m_f, maxJerkU_mps3_f, maxAccUp_mps2_f, maxAccDown_mps2_f, ...
        maxVelUp_mps_f, maxVelDown_mps_f, verticalAcceptanceRadius_m_f, smallValue_f);

    posErrorU_m_f = curWpNEU_m_f(3) - trajPosStateNEU_m_f(3);
    posVelSpU_mps_f = single(0.0);

    if abs(posErrorU_m_f) > smallValue_f
        posVelSpU_mps_f = sign(posErrorU_m_f) * maxAllowedSpeedU_mps_f;
    end

    if velUValid_b
        rawVelSpNEU_mps_f(3) = rawVelSpNEU_mps_f(3) + posVelSpU_mps_f;
    else
        rawVelSpNEU_mps_f(3) = posVelSpU_mps_f;
    end

else
    % 不处理，直接使用前馈速度
end

% 位置速度和速度前馈相加后，统一执行最终性能包线保护。
rawVelSpNEU_mps_f(1:2) = limit_vector_2d(rawVelSpNEU_mps_f(1:2), maxVelNE_mps_f, smallValue_f);     % 超长放缩
rawVelSpNEU_mps_f(3) = constrain_scalar(rawVelSpNEU_mps_f(3), -maxVelDown_mps_f, maxVelUp_mps_f);

%% 选择当前垂向整套约束
% NEU中U向上为正：rawVelSpU>0选择爬升约束，rawVelSpU<0选择下降约束。
if rawVelSpNEU_mps_f(3) > smallValue_f
    selectedUConstraintModeState_i8 = int8(1);
elseif rawVelSpNEU_mps_f(3) < -smallValue_f
    selectedUConstraintModeState_i8 = int8(-1);
else
    % 保持上一周期所选模式，使停车S曲线沿用进入停车前的整套参数。
end

if selectedUConstraintModeState_i8 > int8(0)
    selectedMaxAccU_mps2_f = maxAccUp_mps2_f;
    selectedMaxVelU_mps_f = maxVelUp_mps_f;
elseif selectedUConstraintModeState_i8 < int8(0)
    selectedMaxAccU_mps2_f = maxAccDown_mps2_f;
    selectedMaxVelU_mps_f = maxVelDown_mps_f;
else
    selectedMaxAccU_mps2_f = min(maxAccUp_mps2_f, maxAccDown_mps2_f);
    selectedMaxVelU_mps_f = min(maxVelUp_mps_f, maxVelDown_mps_f);
end

axisMaxAccPlanNEU_mps2_f = single([maxAccNE_mps2_f; maxAccNE_mps2_f; selectedMaxAccU_mps2_f]);
axisMaxVelPlanNEU_mps_f = single([maxVelNE_mps_f; maxVelNE_mps_f; selectedMaxVelU_mps_f]);

%% 计算三轴公共时间拉伸系数
% 水平：只有虚拟轨迹处于实际飞机运动前方时才进行时间拉伸。
timeStretchNE_f = single(1.0);
droneToTrajNE_m_f = trajPosStateNEU_m_f(1:2) - curPosNEU_m_f(1:2);
trajSpeedNE_mps_f = norm(trajVelStateNEU_mps_f(1:2));
trajectoryAheadNE_b = trajSpeedNE_mps_f > smallValue_f && dot(droneToTrajNE_m_f, trajVelStateNEU_mps_f(1:2)) > single(0.0);

if trajectoryAheadNE_b
    normalizedErrorNE_f = norm(droneToTrajNE_m_f) / maxTrajErrorNE_m_f;
    timeStretchNE_f = single(1.0) - constrain_scalar(normalizedErrorNE_f, single(0.0), single(1.0));
end

% 垂向：误差方向与轨迹速度方向一致，说明虚拟轨迹处于实际飞机前方。
timeStretchU_f = single(1.0);
droneToTrajU_m_f = trajPosStateNEU_m_f(3) - curPosNEU_m_f(3);
trajectoryAheadU_b = abs(trajVelStateNEU_mps_f(3)) > smallValue_f && droneToTrajU_m_f * trajVelStateNEU_mps_f(3) > single(0.0);

if trajectoryAheadU_b
    normalizedErrorU_f = abs(droneToTrajU_m_f) / maxTrajErrorU_m_f;
    timeStretchU_f = single(1.0) - constrain_scalar(normalizedErrorU_f, single(0.0), single(1.0));
end

% 三轴必须使用同一个有效时间推进，否则会破坏同步后的T1/T2/T3关系。
timeStretchNEU_f = min(timeStretchNE_f, timeStretchU_f);

%% 根据当前状态和本周期原始速度目标规划S曲线
trajVelSpNEU_mps_f = single(zeros(3,1));
trajDirectionNEU_f = single(zeros(3,1));
trajT1NEU_s_f = single(zeros(3,1));
trajT2NEU_s_f = single(zeros(3,1));
trajT3NEU_s_f = single(zeros(3,1));

for axisIdx_i = 1:3
    [trajVelSpNEU_mps_f(axisIdx_i), trajDirectionNEU_f(axisIdx_i), ...
        trajT1NEU_s_f(axisIdx_i), trajT2NEU_s_f(axisIdx_i), trajT3NEU_s_f(axisIdx_i)] = ...
        update_axis_durations(trajAccStateNEU_mps2_f(axisIdx_i), trajVelStateNEU_mps_f(axisIdx_i), rawVelSpNEU_mps_f(axisIdx_i), axisMaxVelPlanNEU_mps_f(axisIdx_i), ...
        axisMaxAccPlanNEU_mps2_f(axisIdx_i), axisMaxJerkNEU_mps3_f(axisIdx_i), smallValue_f);
end

%% N/E/U三轴时间同步
[trajT1NEU_s_f, trajT2NEU_s_f, trajT3NEU_s_f] = synchronize_trajectory_time_neu(trajT1NEU_s_f, trajT2NEU_s_f, trajT3NEU_s_f, trajAccStateNEU_mps2_f, trajVelStateNEU_mps_f, ...
trajVelSpNEU_mps_f, trajDirectionNEU_f, axisMaxAccPlanNEU_mps2_f, axisMaxJerkNEU_mps3_f, smallValue_f);

%% 用本周期刚得到的同步S曲线推进dt，并保存最小物理状态
trajJerkNEU_mps3_f = single(zeros(3,1));

for axisIdx_i = 1:3
    [trajJerkNEU_mps3_f(axisIdx_i), trajAccStateNEU_mps2_f(axisIdx_i), trajVelStateNEU_mps_f(axisIdx_i), trajPosStateNEU_m_f(axisIdx_i)] = ...
        update_trajectory_axis(trajAccStateNEU_mps2_f(axisIdx_i), trajVelStateNEU_mps_f(axisIdx_i), trajPosStateNEU_m_f(axisIdx_i), trajT1NEU_s_f(axisIdx_i), trajT2NEU_s_f(axisIdx_i), ...
        trajT3NEU_s_f(axisIdx_i), axisMaxJerkNEU_mps3_f(axisIdx_i), trajDirectionNEU_f(axisIdx_i), dtEff_s_f, timeStretchNEU_f);
end

%% 输出本周期推进后的轨迹状态
trajPosNEU_m_f = trajPosStateNEU_m_f;
trajVelNEU_mps_f = trajVelStateNEU_mps_f;
trajAccNEU_mps2_f = trajAccStateNEU_mps2_f;

end

function maxAllowedSpeedU_mps_f = get_max_z_speed_handle(trajPosU_m_f, curWpU_m_f, nextWpU_m_f, maxJerkU_mps3_f, maxAccUp_mps2_f, maxAccDown_mps2_f, ...
    maxVelUp_mps_f, maxVelDown_mps_f, verticalAcceptanceRadius_m_f, smallValue_f)
%#codegen
%
% 根据位置生成速度目标的方向，选择同方向轨迹所使用的整套加速度约束。
% 选中后，get_max_z_speed和后续S曲线均把该值作为对称加速度幅值。
% 不能因为爬升末段需要负加速度刹车，就切换为下降轨迹约束。

posErrorU_m_f = curWpU_m_f - trajPosU_m_f;

if posErrorU_m_f > smallValue_f
    maxAccSelectedU_mps2_f = maxAccUp_mps2_f;
elseif posErrorU_m_f < -smallValue_f
    maxAccSelectedU_mps2_f = maxAccDown_mps2_f;
else
    % 当前高度误差很小时，根据下一航段速度目标方向选择约束。
    nextSegmentDeltaU_m_f = nextWpU_m_f - curWpU_m_f;

    if nextSegmentDeltaU_m_f > smallValue_f
        maxAccSelectedU_mps2_f = maxAccUp_mps2_f;
    elseif nextSegmentDeltaU_m_f < -smallValue_f
        maxAccSelectedU_mps2_f = maxAccDown_mps2_f;
    else
        maxAccSelectedU_mps2_f = min(maxAccUp_mps2_f, maxAccDown_mps2_f);
    end
end

maxAllowedSpeedU_mps_f = get_max_z_speed(trajPosU_m_f, curWpU_m_f, nextWpU_m_f, maxJerkU_mps3_f, maxAccSelectedU_mps2_f, maxVelUp_mps_f, ...
    maxVelDown_mps_f, verticalAcceptanceRadius_m_f, smallValue_f);

end

function [crossingPointNEU_m_f, targetSpeedNE_mps_f, previousMaxSpeedNEOut_mps_f] = get_xy_guidance_constraints_handle(trajPosNEU_m_f, trajVelNEU_mps_f, waypointsNEU_m_f, ...
    isHoverWp_b, cruiseSpeedNE_mps_f, maxJerkNE_mps3_f, maxAccNE_mps2_f, horizonAptRadius_m_f, minLookaheadDist_m_f, turnMinSpeed_mps_f, ...
    turnCosThreshold_f, previousMaxSpeedNEIn_mps_f, smallValue_f)
%#codegen
%
% 统一生成3D和2D位置分支共用的水平追踪点及允许速度。
% isHoverWp_b和前倾转换均直接追踪当前航点，其余航段允许使用crossing point。

curWpNEU_m_f = waypointsNEU_m_f(:,2);

if isHoverWp_b
    crossingPointNEU_m_f = curWpNEU_m_f;
    distanceToTargetNE_m_f = norm(curWpNEU_m_f(1:2) - trajPosNEU_m_f(1:2));
    maxStopSpeedNE_mps_f = compute_max_speed_from_distance(maxJerkNE_mps3_f, maxAccNE_mps2_f, distanceToTargetNE_m_f, single(0.0), smallValue_f);
    targetSpeedNE_mps_f = min(cruiseSpeedNE_mps_f, maxStopSpeedNE_mps_f);

else
    crossingPointNEU_m_f = get_crossing_point(trajPosNEU_m_f, trajVelNEU_mps_f, waypointsNEU_m_f, horizonAptRadius_m_f, minLookaheadDist_m_f, ...
        turnMinSpeed_mps_f, turnCosThreshold_f, smallValue_f);
    targetSpeedNE_mps_f = cruiseSpeedNE_mps_f;
end

turning_b = is_turning(trajPosNEU_m_f, trajVelNEU_mps_f, curWpNEU_m_f, horizonAptRadius_m_f, turnMinSpeed_mps_f, turnCosThreshold_f, smallValue_f);

if ~isHoverWp_b && turning_b
    % 在转弯过程中不允许本周期目标速度高于转弯前锁存值。
    % 若在运动中复位导致锁存值尚未建立，则先用当前候选值初始化。
    if previousMaxSpeedNEIn_mps_f > smallValue_f
        targetSpeedNE_mps_f = min(previousMaxSpeedNEIn_mps_f, targetSpeedNE_mps_f);
    end

    previousMaxSpeedNEOut_mps_f = targetSpeedNE_mps_f;
else
    previousMaxSpeedNEOut_mps_f = targetSpeedNE_mps_f;
end

end

function outputNEU_mps_f = clamp_to_xy_norm(inputNEU_mps_f, maxNormNE_mps_f, accuracy_mps_f, floatEpsilon_f)
%#codegen
%
% 1. 一般超限时按同一比例缩放整个NEU向量，保持三维方向不变；
% 2. 当水平上限和当前水平模长均小于accuracy时，只缩放NE分量，
%    避免微小水平数值误差把有效U速度一并缩小；

outputNEU_mps_f = inputNEU_mps_f;
normNEU_mps_f = norm(inputNEU_mps_f(1:2));
scaleFactor_f = single(1.0);

if normNEU_mps_f > floatEpsilon_f
    scaleFactor_f = maxNormNE_mps_f / normNEU_mps_f;
end

if scaleFactor_f < single(1.0)
    if maxNormNE_mps_f < accuracy_mps_f && normNEU_mps_f < accuracy_mps_f
        outputNEU_mps_f(1:2) = inputNEU_mps_f(1:2) * scaleFactor_f;
    else
        outputNEU_mps_f = inputNEU_mps_f * scaleFactor_f;
    end
end

end

function outputNEU_mps_f = clamp_to_u_norm(inputNEU_mps_f, maxNormU_mps_f, accuracy_mps_f, floatEpsilon_f)
%#codegen
%
% 1. 一般超限时按同一比例缩放整个NEU向量，保持三维方向不变；
% 2. 当垂向上限和当前垂向模长均小于accuracy时，只缩放U分量，
%    避免微小垂向数值误差把有效NE速度一并缩小。

outputNEU_mps_f = inputNEU_mps_f;
absSpeedU_mps_f = abs(inputNEU_mps_f(3));
scaleFactor_f = single(1.0);

if absSpeedU_mps_f > floatEpsilon_f
    scaleFactor_f = maxNormU_mps_f / absSpeedU_mps_f;
end

if scaleFactor_f < single(1.0)
    if maxNormU_mps_f < accuracy_mps_f && absSpeedU_mps_f < accuracy_mps_f
        outputNEU_mps_f(3) = inputNEU_mps_f(3) * scaleFactor_f;
    else
        outputNEU_mps_f = inputNEU_mps_f * scaleFactor_f;
    end
end

end

== matlab function GuidanceLaw/Subsystem/wpMssnHandle/GuiLaw/yawGuidance/yawGuidance ==
  data: yawCmd_deg_f output; segMssnType_u8 input; curWp_struct input; preWp_struct input; nextWp_struct input; nav_struct input; trajVelNEU_mps_f input; isHoverPosReach_b input; yawHold_deg_f input; curPosNEU_m_f input; yawTrajectory_deg_f output
function [yawCmd_deg_f, yawTrajectory_deg_f] = mcTrajFlagManager(segMssnType_u8, curWp_struct, preWp_struct, nextWp_struct, nav_struct, trajVelNEU_mps_f, isHoverPosReach_b, yawHold_deg_f, curPosNEU_m_f)
%#codegen
%
% 旋翼/前倾转换阶段偏航角指令生成
%
% 功能：
% 1. 垂直起飞位置到达前保持进入任务时的偏航角；
% 2. 垂直起飞位置到达后，根据下一航点偏航类型调整航向；
% 3. 减速悬停位置到达前，根据当前航点偏航类型生成偏航角；
% 4. 减速悬停位置到达后，根据下一航点偏航类型生成偏航角；
% 5. 快速过点阶段始终跟随轨迹水平速度方向；
% 6. 航向对准模式下，运动阶段跟随轨迹速度方向；
% 7. 航点指定模式下，使用相应航点指定的偏航角；
% 8. 指向航点模式下，根据飞机当前位置和目标航点计算偏航角；
% 9. 垂直着陆阶段保持进入着陆任务时的偏航角；
% 10. 前倾转换阶段对准当前转换航段preWp -> curWp；
% 11. 轨迹水平速度过小时使用当前实际航向；
% 12. 未定义的航段任务类型保持当前实际航向。
%
% curWp_struct.yawType_u8、nextWp_struct.yawType_u8
%   0：航向对准
%   1：航点指定
%   2：指向航点

%% 常量

rad2deg_f = single(57.29577951308232);

%% 基本输入量

curYaw_deg_f = cldWrap180(nav_struct.yaw_deg_f);
yawHold_deg_f = cldWrap180(yawHold_deg_f);

curYawType_u8 = curWp_struct.yawType_u8;
nextYawType_u8 = nextWp_struct.yawType_u8;

curSpecifiedYaw_deg_f = cldWrap180(curWp_struct.yaw_deg_f);
nextSpecifiedYaw_deg_f = cldWrap180(nextWp_struct.yaw_deg_f);

trajVelN_mps_f = trajVelNEU_mps_f(1);
trajVelE_mps_f = trajVelNEU_mps_f(2);

curFastWp = curWp_struct.fastWp_b;
%% 计算轨迹切向偏航角

trajSpeedSq_m2ps2_f = sqrt(trajVelN_mps_f * trajVelN_mps_f + trajVelE_mps_f * trajVelE_mps_f);

if trajSpeedSq_m2ps2_f >= single(0.1)

    yawTrajectory_deg_f = single(atan2(trajVelE_mps_f, trajVelN_mps_f)) * rad2deg_f;
    yawTrajectory_deg_f = cldWrap180(yawTrajectory_deg_f);

else
    % 轨迹水平速度过小时，速度方向不可靠。
    yawTrajectory_deg_f = curYaw_deg_f;

end

%% 计算飞机当前位置指向当前航点的偏航角

curWpDirN_m_f = curWp_struct.posN_m_f - curPosNEU_m_f(1);
curWpDirE_m_f = curWp_struct.posE_m_f - curPosNEU_m_f(2);

yawPosToCurWp_deg_f = calcHorizonYaw(curWpDirN_m_f, curWpDirE_m_f, curYaw_deg_f);

%% 计算飞机当前位置指向下一航点的偏航角

nextWpDirN_m_f = nextWp_struct.posN_m_f - curPosNEU_m_f(1);
nextWpDirE_m_f = nextWp_struct.posE_m_f - curPosNEU_m_f(2);

yawPosToNextWp_deg_f = calcHorizonYaw(nextWpDirN_m_f, nextWpDirE_m_f, curYaw_deg_f);

%% 计算当前航点到下一航点的航段偏航角

nextPathN_m_f = nextWp_struct.posN_m_f - curWp_struct.posN_m_f;
nextPathE_m_f = nextWp_struct.posE_m_f - curWp_struct.posE_m_f;

yawNextPath_deg_f = calcHorizonYaw(nextPathN_m_f, nextPathE_m_f, curYaw_deg_f);

%% 计算上一航点到当前航点的航段偏航角

currentPathN_m_f = curWp_struct.posN_m_f - preWp_struct.posN_m_f;
currentPathE_m_f = curWp_struct.posE_m_f - preWp_struct.posE_m_f;

yawCurrentPath_deg_f = calcHorizonYaw(currentPathN_m_f, currentPathE_m_f, yawHold_deg_f);

%% 计算悬停位置到达后的偏航角

if nextYawType_u8 == uint8(0)

    % 航向对准：
    % 对准curWp -> nextWp航段。
    yawAfterHover_deg_f = yawNextPath_deg_f;

elseif nextYawType_u8 == uint8(1)

    % 航点指定：
    % 使用下一航点指定的偏航角。
    yawAfterHover_deg_f = nextSpecifiedYaw_deg_f;

elseif nextYawType_u8 == uint8(2)

    % 指向航点：
    % 从当前位置指向下一航点。
    yawAfterHover_deg_f = yawPosToNextWp_deg_f;

else

    % 偏航类型无效时保持当前实际航向。
    yawAfterHover_deg_f = curYaw_deg_f;

end

%% 根据航段任务类型生成偏航角指令

% ==============================================================
% 1. 旋翼垂直起飞
% ==============================================================

if segMssnType_u8 == uint8(1)

    if isHoverPosReach_b

        % 到达垂直起飞目标位置后，
        % 根据下一航点的偏航类型调整航向。
        yawTarget_deg_f = yawAfterHover_deg_f;

    else

        % 垂直起飞过程中保持进入任务时的偏航角。
        yawTarget_deg_f = yawHold_deg_f;

    end


% ==============================================================
% 2. 旋翼直线
% ==============================================================

elseif segMssnType_u8 == uint8(2)

    if curFastWp == false

        if isHoverPosReach_b
    
            % 到达当前悬停位置后，
            % 根据下一航点的偏航类型调整航向。
            yawTarget_deg_f = yawAfterHover_deg_f;
    
        else
    
            % 尚未到达当前悬停位置，
            % 根据当前航点的偏航类型生成偏航角。
    
            if curYawType_u8 == uint8(0)
    
                % 航向对准：跟随轨迹水平速度方向。
                yawTarget_deg_f = yawTrajectory_deg_f;
    
            elseif curYawType_u8 == uint8(1)
    
                % 航点指定：使用当前航点指定偏航角。
                yawTarget_deg_f = curSpecifiedYaw_deg_f;
    
            elseif curYawType_u8 == uint8(2)
    
                % 指向航点：从当前位置指向当前目标航点。
                yawTarget_deg_f = yawPosToCurWp_deg_f;
    
            else
    
                % 偏航类型无效时保持当前实际航向。
                yawTarget_deg_f = curYaw_deg_f;
    
            end
    
        end
    else
        % 快速过点不执行航点指定和指向航点策略，
        % 始终跟随轨迹水平速度方向。
        yawTarget_deg_f = yawTrajectory_deg_f;
    end

% ==============================================================
% 4. 旋翼垂直着陆
% ==============================================================

elseif segMssnType_u8 == uint8(3)

    % 垂直下降过程中锁定进入着陆任务时的偏航角。
    yawTarget_deg_f = yawHold_deg_f;


% ==============================================================
% 5. 旋翼前倾转换（是否要按照L1的导引航向？）
% ==============================================================

elseif segMssnType_u8 == uint8(4)

    % 当前转换航段定义为preWp -> curWp，
    % 前倾转换阶段对准当前转换航段。
    yawTarget_deg_f = yawCurrentPath_deg_f;


% ==============================================================
% 其他无效任务类型
% ==============================================================

else

    yawTarget_deg_f = curYaw_deg_f;

end

%% 输出

yawCmd_deg_f = cldWrap180(yawTarget_deg_f);

end

== matlab function GuidanceLaw/Subsystem/wpMssnHandle/GuiLaw/mcSpdGuidance/mcTrajFlagManager ==
  data: curWp_struct input; isHoverWp_b output; forceStop_b output; posVelValid_vec output; takeoffSwitchKp_f input; climbRate_mps_f input; nav_struct input; maxSwitchAlt_m_f input; segMssnType_u8 input; velSpNEU_mps_vec output; lowHeight_m_f input; highHeight_m_f input; minDescentRate_mps_f input; maxDescentRate_mps_f input; fixedDescentRate_mps_f input; curPosU_m_f input; preWp_struct input
function [isHoverWp_b, forceStop_b, posVelValid_vec, velSpNEU_mps_vec] = mcTrajFlagManager(curWp_struct, takeoffSwitchKp_f, climbRate_mps_f, nav_struct, maxSwitchAlt_m_f, segMssnType_u8,...
    lowHeight_m_f, highHeight_m_f, minDescentRate_mps_f, maxDescentRate_mps_f, fixedDescentRate_mps_f, curPosU_m_f, preWp_struct)
%#codegen
%
% 功能：
% 根据导引律选择结果、飞行阶段和当前航点类型，统一生成旋翼轨迹生成器使用的使能标志。

% posVelValid_vec = [posNEValid_b;velNEValid_b;posUValid_b;velUValid_b]
%   posNEValid  velNEValid   NE模式
%       1           0        纯位置
%       0           1        纯速度
%       1           1        位置 + 速度前馈
%       0           0        NE目标无效
%
%   posUValid   velUValid    U模式
%       1           0        纯位置
%       0           1        纯速度
%       1           1        位置 + 速度前馈
%       0           0        U目标无效

% 典型组合：
% 1. 航线位置飞行：
%       posNEValid=1, velNEValid=0
%       posUValid =1, velUValid =0
%
% 3. 起飞初期“水平位置 + 初始固定爬升速度”：
%       posNEValid=1, velNEValid=0
%       posUValid =0, velUValid =1

forceStop_b = false;
posVelValid_vec = uint8(zeros(4,1));

curWpU_m_f = curWp_struct.posU_m_f;
preWpU_m_f = preWp_struct.posU_m_f;
curhag_m_f = nav_struct.hag_m_f;
curhagValid_m_f = nav_struct.hagValid_b;
curFastWp_b = curWp_struct.fastWp_b;

velSpNEU_mps_vec = single(zeros(3,1));

%% 根据当前旋翼航段任务类型，设置轨迹生成器模式
% posVelValid_vec = [posNEValid_b;velNEValid_b;posUValid_b;velUValid_b]
% 0：无效，1：旋翼垂直起飞，2：旋翼直线，3：旋翼垂直降落，4：旋翼前倾，5：固定翼后倾，6：固定翼直线，7：固定翼圆弧
% 旋翼垂直起飞
if segMssnType_u8 == uint8(1)

    deltaAlt_m_f = max(curWpU_m_f - preWpU_m_f,single(0));
    switchHeight_m_f = min(maxSwitchAlt_m_f, takeoffSwitchKp_f * deltaAlt_m_f);
    climbedHeight_m_f = max(curPosU_m_f - preWpU_m_f,single(0));
    switchToPos_b = climbedHeight_m_f >= switchHeight_m_f;

    if switchToPos_b
        % NE位置 + U位置
        posVelValid_vec(1) = uint8(1);
        posVelValid_vec(3) = uint8(1);
    else
        % NE位置 + U速度
        posVelValid_vec(1) = uint8(1);
        posVelValid_vec(4) = uint8(1);
        velSpNEU_mps_vec(3) = climbRate_mps_f;
    end

    % 水平位置需要稳定在起飞点。
    isHoverWp_b = true;

% 旋翼直线
elseif segMssnType_u8 == uint8(2)
    % NE位置 + U位置
    posVelValid_vec(1) = uint8(1);
    posVelValid_vec(3) = uint8(1);
    if curFastWp_b == false
        % 减速悬停
        isHoverWp_b = true;
    else
        % 快速过点
        isHoverWp_b = false;
    end

% 旋翼垂直着陆
elseif segMssnType_u8 == uint8(3)

    % NE位置 + U速度
    posVelValid_vec(1) = uint8(1);
    posVelValid_vec(4) = uint8(1);

    velSpNEU_mps_vec(3) = descentRateGuidance(curhag_m_f, curhagValid_m_f, lowHeight_m_f, highHeight_m_f, minDescentRate_mps_f, maxDescentRate_mps_f, fixedDescentRate_mps_f);

    % 垂直着陆
    isHoverWp_b = true;

% % 旋翼前倾过渡，以固定翼方式处理
% elseif segMssnType_u8 == uint8(4)
% 
%     % NE位置 + U位置
%     posVelValid_vec(1) = uint8(1);
%     posVelValid_vec(3) = uint8(1);
% 
%     % 前倾过渡
%     isHoverWp_b = false;
else
    % 这种情况不会出现，以防万一强制刹停
    forceStop_b = true;
    isHoverWp_b = false;
end

end

function descentVelCmd_mps_f = descentRateGuidance(curHag_m_f, hagValid_b, lowHeight_m_f, highHeight_m_f, minDescentRate_mps_f, maxDescentRate_mps_f, fixedDescentRate_mps_f)
%#codegen
%
% 功能：
% 根据当前相对高度分段生成着陆下沉速度指令。
%
% 输入：
% curHag_m_f              当前相对高度，m
% hagValid_b              高度有效标志
% lowHeight_m_f           低高度分界值，m
% highHeight_m_f          高高度分界值，m
% minDescentRate_mps_f    最小下沉率幅值，m/s
% maxDescentRate_mps_f    最大下沉率幅值，m/s
% fixedDescentRate_mps_f  固定下沉率幅值，m/s
%
% 输出：
% descentVelCmd_mps_f     垂向速度指令，m/s，向上为正
%
% 分段逻辑：
% 1. 高度无效：固定输出 -0.6 m/s；
% 2. h <= lowHeight：使用最小下沉率；
% 3. h >= highHeight：使用最大下沉率；
% 4. 中间高度：线性插值。

%% 高度失效保护

if hagValid_b == false
    descentVelCmd_mps_f = -fixedDescentRate_mps_f;
    return;
end

%% 参数保护

minDescentRate_mps_f = max(minDescentRate_mps_f, 0.0);
maxDescentRate_mps_f = max(maxDescentRate_mps_f, minDescentRate_mps_f);

if highHeight_m_f <= lowHeight_m_f
    descentVelCmd_mps_f = -minDescentRate_mps_f;
    return;
end

%% 分段计算下沉率幅值

if curHag_m_f <= lowHeight_m_f
    descentRate_mps_f = minDescentRate_mps_f;

elseif curHag_m_f >= highHeight_m_f
    descentRate_mps_f = maxDescentRate_mps_f;

else
    heightRatio_f = (curHag_m_f - lowHeight_m_f) / (highHeight_m_f - lowHeight_m_f);

    descentRate_mps_f = minDescentRate_mps_f + heightRatio_f * (maxDescentRate_mps_f - minDescentRate_mps_f);
end

%% 转换为向上为正的垂向速度指令

descentVelCmd_mps_f = -descentRate_mps_f;

end

== stateflow chart GuidanceLaw/Subsystem/wpMssnHandle/WpUpdate/WaypointManager ==
  state EXECUTE
    entry:
    segSwitch_b = true;
    routeActive_b = true;
    routeComplete_b = false;
    if route_struct(curWpIdx_u8 - uint8(1)).wpType_u8 == WP_TYPE.FW_CIR_WP && ...
    route_struct(curWpIdx_u8).wpType_u8 == WP_TYPE.FW_LINE_WP
    curWpIdx_u8 = curWpIdx_u8 + uint8(1);
    if curWpIdx_u8 >= validWpNum_u8
    segSwitch_b = false;
    routeActive_b = false;
    routeComplete_b = true;
    end
    end
    during:
    segSwitch_b = false;
  state NO_ROUTE
    entry:
    curWpIdx_u8 = uint8(0);
    segSwitch_b = false;
    routeActive_b = false;
    routeComplete_b = false;
  note: 着陆完成判定需要依靠外部着陆标志
  state COMPLETE
    entry:
    segSwitch_b = false;
    routeActive_b = false;
    routeComplete_b = true;
  (default) -> (junction 21)
  (junction 21) -> EXECUTE [order 1] : [routeUpdate_b && validWpNum_u8 >= uint8(2)]{curWpIdx_u8 = uint8(2);}
  EXECUTE -> EXECUTE [order 1] : [routeUpdate_b && validWpNum_u8 >= uint8(2)]{curWpIdx_u8 = uint8(2);}
  (junction 21) -> NO_ROUTE [order 2]
  EXECUTE -> NO_ROUTE [order 2] : [routeUpdate_b && validWpNum_u8 < uint8(2)]
  EXECUTE -> EXECUTE [order 3] : [~routeUpdate_b && wpCompletePulse_b && curWpIdx_u8 < validWpNum_u8]{curWpIdx_u8 = curWpIdx_u8 + uint8(1);}
  NO_ROUTE -> EXECUTE : [routeUpdate_b && validWpNum_u8 >= uint8(2)]{curWpIdx_u8 = uint8(2);}
  COMPLETE -> NO_ROUTE [order 2] : [routeUpdate_b && validWpNum_u8 < uint8(2)]
  COMPLETE -> EXECUTE [order 1] : [routeUpdate_b && validWpNum_u8 >= uint8(2)]{curWpIdx_u8 = uint8(2);}
  EXECUTE -> COMPLETE [order 4] : [~routeUpdate_b && wpCompletePulse_b && curWpIdx_u8 >= validWpNum_u8]
  data: routeUpdate_b input boolean; wpCompletePulse_b input boolean; validWpNum_u8 input uint8; curWpIdx_u8 output uint8; segSwitch_b output boolean; routeActive_b output boolean; routeComplete_b output boolean; route_struct input
